simulink model "Simulateur_palan"  (R2024b)
settings: Solver=ode4  StartTime=0.0  StopTime=20  RelTol=1e-3
values from neighbouring files (symbols this model uses):
  A = [   0   1    0   0 ... (first row only)    [ETAT_PAL_IDENT.m]    (also in Essai_boucle_ouverte.mat = [0 0 0 0 1 -7.87878787879 0 78.7878787879 0 0 0 -98.1 ... (1)
  B = [   0 ... (first row only)    [ETAT_PAL_IDENT.m]    (also in Essai_boucle_ouverte.mat = [0 2.52121212121 0 -25.2121212121])
  Kr = [0.1 0 0 0]    [Essai_boucle_ouverte.mat]    (also in labo6_simulation.m = [k 0 0 0])
  L = 0.1    [ETAT_PAL_IDENT.m]    (also in Essai_boucle_ouverte.mat; labo6_simulation.m = 1; p1_cre_18V_droite_0m.mat = 0; p1_cre_18V_droite_1m.mat = 1)
  xd = [0.5 0 0 0]    [Essai_boucle_ouverte.mat]    (also in labo6_simulation.m = [0.1 0 0 0]')
settings Model: Creator=Ale  LastModifiedBy=Ale

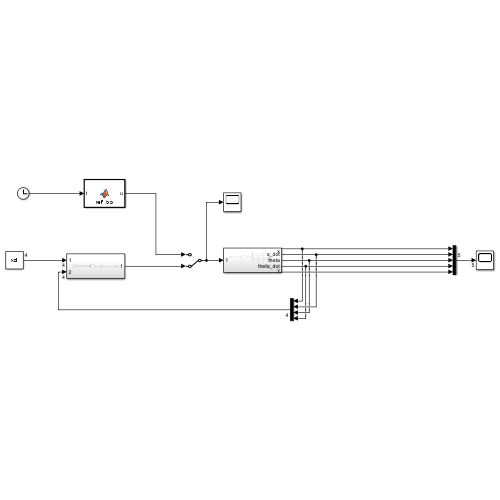
[thumbnail: Simulink's stored preview of the top-level diagram]
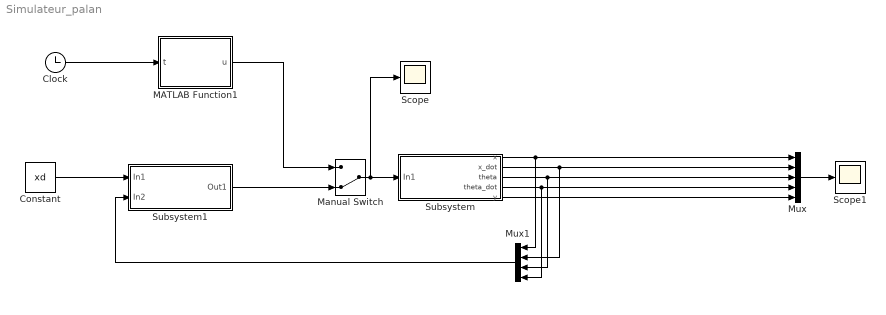
== system Simulateur_palan ==
  Clock : Clock
  Constant : Constant  Value=xd
  MATLAB Function1 : MATLAB Function  TreatAsAtomicUnit=on
  Manual Switch : ManualSwitch  CurrentSetting=0
  Mux : Mux  Inputs=5
  Mux1 : Mux
  Scope : Scope
  Scope1 : Scope
  Subsystem : Subsystem
  Subsystem1 : Subsystem
  wires:
  Manual Switch/1 -> Scope/1, Subsystem/1(In1)
  Subsystem/1(x) -> Mux1/1, Mux/1
  Subsystem/2(x_dot) -> Mux1/2, Mux/2
  Subsystem/3(theta) -> Mux1/3, Mux/3
  Subsystem/4(theta_dot) -> Mux1/4, Mux/4
  Subsystem/5(y) -> Mux/5
  Mux/1 -> Scope1/1
  MATLAB Function1/1(u) -> Manual Switch/1
  Constant/1 -> Subsystem1/1(In1)
  Mux1/1 -> Subsystem1/2(In2)
  Subsystem1/1(Out1) -> Manual Switch/2
  Clock/1 -> MATLAB Function1/1(t)

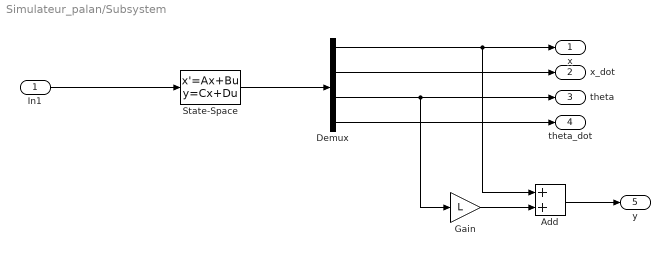
== system Simulateur_palan/Subsystem ==
  In1 : Inport
  Add : Sum
  Demux : Demux
  Gain : Gain  Gain=L
  State-Space : StateSpace  A=A  B=B  C=[1 0 0 0;0 1 0 0; 0 0 1 0; 0 0 0 1]  D=[0;0;0;0]  InitialCondition=0
  x : Outport
  x_dot : Outport  Port=2
  theta : Outport  Port=3
  theta_dot : Outport  Port=4
  y : Outport  Port=5
  wires:
  In1/1 -> State-Space/1
  State-Space/1 -> Demux/1
  Demux/2 -> x_dot/1
  Demux/1 -> x/1, Add/1
  Demux/4 -> theta_dot/1
  Demux/3 -> theta/1, Gain/1
  Gain/1 -> Add/2
  Add/1 -> y/1

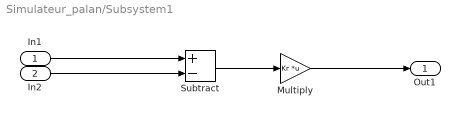
== system Simulateur_palan/Subsystem1 ==
  In1 : Inport
  In2 : Inport  Port=2
  Multiply : Gain  Gain=Kr  Multiplication=Matrix(K*u)
  Subtract : Sum  Inputs=+-
  Out1 : Outport
  wires:
  In1/1 -> Subtract/1
  In2/1 -> Subtract/2
  Subtract/1 -> Multiply/1
  Multiply/1 -> Out1/1

== matlab function Simulateur_palan/MATLAB Function1 ==
  data: t input; u output
function u = ref_bo(t)

if t<=0 
u = 0 ;

elseif (t>0 && t<=1)
u=1;

elseif (t>1 && t<=2)
u=-1;

else 
u=0;

end
